simulink model "A9_Code_preparation"  (R2026a)
settings: Solver=FixedStepDiscrete  StopTime=t_final  FixedStep=Ts
InitFcn:
  | A8_init_TCLab_SIMC
undefined symbols (not defined in the file): den_Gp_d, dspblkCoreblockFVToolHelper, gcbh, N_delay, num_Gp_d, T_amb, T_ref, Ts
settings Model: Creator=jguerrero  LastModifiedBy=jordy

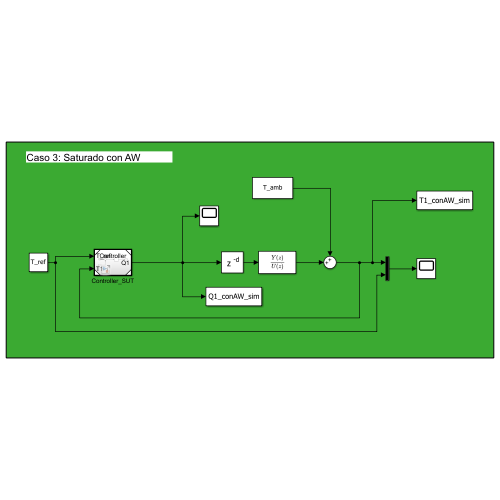
[thumbnail: Simulink's stored preview of the top-level diagram]
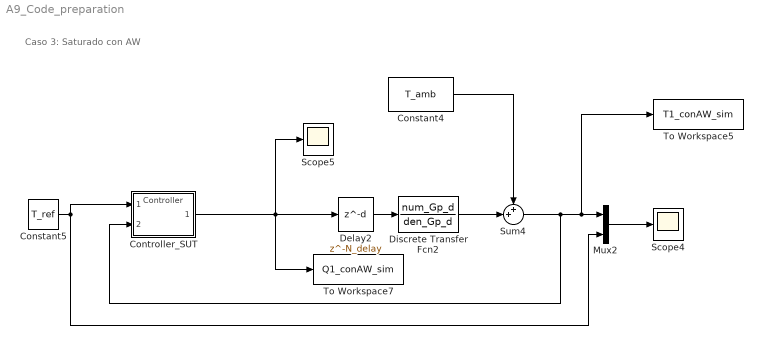
== system A9_Code_preparation ==
  note: Caso 3: Saturado con AW
  Constant4 : Constant  Value=T_amb  SampleTime=Ts
  Constant5 : Constant  Value=T_ref  SampleTime=Ts
  Controller_SUT : ModelReference  ModelNameDialog=Controller  SimulationMode=Normal  ModelReferenceVersion=1.12
  Delay2 : Delay  DelayLength=N_delay  SampleTime=Ts
  Discrete Transfer Fcn2 : DiscreteTransferFcn  LoadFcn=dspblkCoreblockFVToolHelper(gcbh,'load');  Numerator=num_Gp_d  Denominator=den_Gp_d
      settings: CopyFcn=dspblkCoreblockFVToolHelper(gcbh,'copy');  DeleteFcn=dspblkCoreblockFVToolHelper(gcbh,'close');  ModelCloseFcn=dspblkCoreblockFVToolHelper(gcbh,'close');  PreSaveFcn=dspblkCoreblockFVToolHelper(gcbh,'presave');  PostSaveFcn=dspblkCoreblockFVToolHelper(gcbh,'postsave');  CloseFcn=dspblkCoreblockFVToolHelper(gcbh,'close');
  Mux2 : Mux  Inputs=2
  Scope4 : Scope
      settings: ActiveDisplayYMinimum=20.625  ActiveDisplayYMaximum=64.375  DataLoggingVariableName=ScopeData4
  Scope5 : Scope
      settings: ActiveDisplayYMinimum=27.921311930843586  ActiveDisplayYMaximum=96.897632007684052  DataLoggingVariableName=ScopeData5
  Sum4 : Sum  Inputs=++|
  To Workspace5 : ToWorkspace  VariableName=T1_conAW_sim  SaveFormat=Timeseries  SampleTime=-1
  To Workspace7 : ToWorkspace  VariableName=Q1_conAW_sim  SaveFormat=Timeseries  SampleTime=-1
  wires:
  Constant4/1 -> Sum4/1
  Sum4/1 -> Controller_SUT/2, Mux2/1, To Workspace5/1
  Delay2/1 -> Discrete Transfer Fcn2/1
  Discrete Transfer Fcn2/1 -> Sum4/2
  Mux2/1 -> Scope4/1
  Constant5/1 -> Controller_SUT/1, Mux2/2
  Controller_SUT/1 -> Scope5/1, To Workspace7/1, Delay2/1
